simulink model "mod_ook"  (R2024b)
settings: Solver=FixedStepDiscrete  StartTime=0.0  StopTime=1  FixedStep=3.1250000000000001e-05  RelTol=1e-3
model workspace (MAT data in the model file):
  M = 2
  Ts = 0.001
  decalage = 0.00096875
  df_ol = 1
  fc = 4000
  fs = 32000
  gain_ech = 2
  graine = 7
  h_rx = [0.03125 0.03125 0.03125 0.03125 0.03125 0.03125 0.03125 0.03125 0.03125 0.03125 0.03125 0.03125 0.03125 0.03125 0.03125 0.03125 0.03125 0.03125 0.03125 0.03125 0.03125 0.03125 0.03125 0.03125 0.03125 0.03125 0.03125 0.03125 0.03125 0.03125 0.03125 0.03125]
  ordre = 1
  phi_ol = 0.7
  points = [0 2]
  ptsI = [0 1]
  ptsQ = [0 0]
  sigma2 = 0
  sps = 32
  w_boucle = 0.000490873852123
libraries: simulink x1
settings Model: Creator=runner  LastModifiedBy=runner

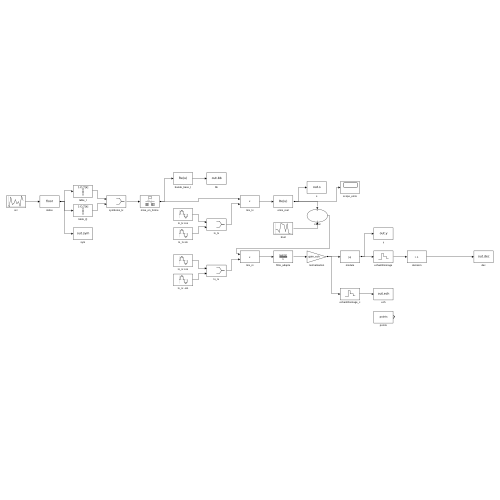
[thumbnail: Simulink's stored preview of the top-level diagram]
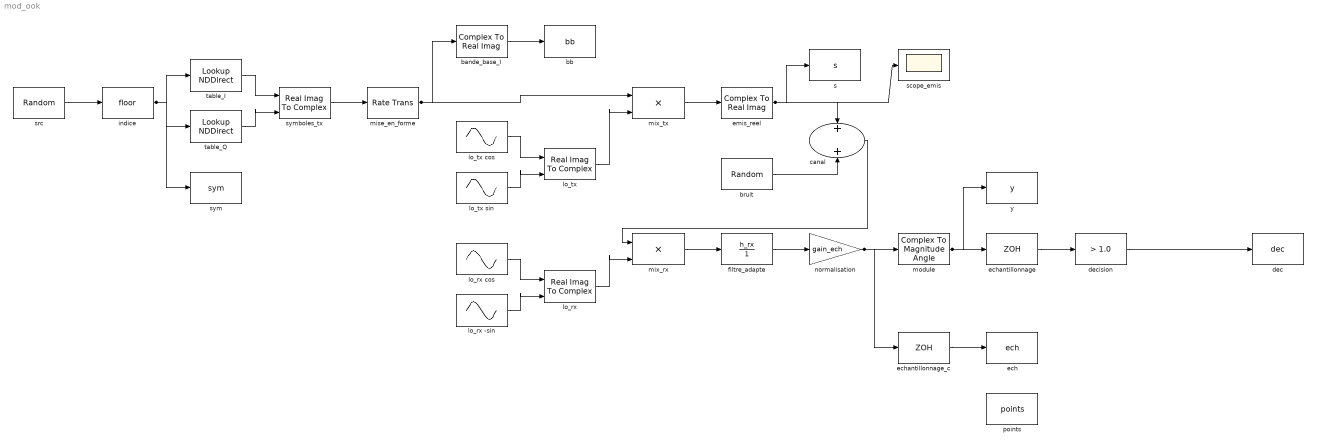
== system mod_ook ==
  bande_base_I : ComplexToRealImag  Output=Real
  bb : ToWorkspace  VariableName=bb  SampleTime=-1
  bruit : RandomNumber  Variance=sigma2  Seed=1  SampleTime=1/fs
  canal : Sum
  dec : ToWorkspace  VariableName=dec  SampleTime=-1
  decision : simulink/Logic and Bit Operations/Compare To Constant  relop=>  const=1.0  OutDataTypeStr=boolean
  ech : ToWorkspace  VariableName=ech  SampleTime=-1
  echantillonnage : ZeroOrderHold  SampleTime=[Ts, decalage]
  echantillonnage_c : ZeroOrderHold  SampleTime=[Ts, decalage]
  emis_reel : ComplexToRealImag  Output=Real
  filtre_adapte : DiscreteFilter  Numerator=h_rx  Denominator=1
  indice : Rounding
  lo_rx : RealImagToComplex
  lo_rx -sin : Sin  Amplitude=-2  Frequency=2*pi*(fc+df_ol)  Phase=phi_ol  SampleTime=1/fs
  lo_rx cos : Sin  Amplitude=2  Frequency=2*pi*(fc+df_ol)  Phase=phi_ol+pi/2  SampleTime=1/fs
  lo_tx : RealImagToComplex
  lo_tx cos : Sin  Frequency=2*pi*fc  Phase=pi/2  SampleTime=1/fs
  lo_tx sin : Sin  Frequency=2*pi*fc  SampleTime=1/fs
  mise_en_forme : RateTransition  OutPortSampleTime=1/fs
  mix_rx : Product
  mix_tx : Product
  module : ComplexToMagnitudeAngle  Output=Magnitude
  normalisation : Gain  Gain=gain_ech
  points : Constant  Value=points
  s : ToWorkspace  VariableName=s  SampleTime=-1
  scope_emis : Scope
  src : UniformRandomNumber  Minimum=0  Maximum=M  Seed=graine  SampleTime=Ts
  sym : ToWorkspace  VariableName=sym  SampleTime=-1
  symboles_tx : RealImagToComplex
  table_I : LookupNDDirect  NumberOfTableDimensions=1  Table=ptsI
  table_Q : LookupNDDirect  NumberOfTableDimensions=1  Table=ptsQ
  y : ToWorkspace  VariableName=y  SampleTime=-1
  wires:
  src/1 -> indice/1
  indice/1 -> table_I/1, table_Q/1, sym/1
  table_I/1 -> symboles_tx/1
  table_Q/1 -> symboles_tx/2
  symboles_tx/1 -> mise_en_forme/1
  mise_en_forme/1 -> bande_base_I/1, mix_tx/1
  bande_base_I/1 -> bb/1
  lo_tx cos/1 -> lo_tx/1
  lo_tx sin/1 -> lo_tx/2
  lo_tx/1 -> mix_tx/2
  mix_tx/1 -> emis_reel/1
  emis_reel/1 -> canal/1, s/1, scope_emis/1
  bruit/1 -> canal/2
  lo_rx cos/1 -> lo_rx/1
  lo_rx -sin/1 -> lo_rx/2
  canal/1 -> mix_rx/1
  lo_rx/1 -> mix_rx/2
  mix_rx/1 -> filtre_adapte/1
  filtre_adapte/1 -> normalisation/1
  normalisation/1 -> module/1, echantillonnage_c/1
  module/1 -> y/1, echantillonnage/1
  echantillonnage_c/1 -> ech/1
  echantillonnage/1 -> decision/1
  decision/1 -> dec/1
